simulink library "ASEToolBox"  (R2025b)
settings: Solver=ode45  StartTime=0.0  StopTime=10.0  RelTol=1e-3  EnableMultiTasking=on
values from neighbouring files (symbols this model uses):
  dt = get_param(gcbh, 'g_output_datatype')    [maskSysComCallbacks_Receive.m]    (also in maskSysComCallbacks_Send.m = get_param(gcbh, 'g_input_datatype'))
undefined symbols (not defined in the file or in its folder): dCx, dCy, dCz, DiscIntNeverNeededParam, Discrete, dmassX, dmassY, dmassZ, dMx, dMy, dMz, dp, dp0, dp1, dp2, dp3, dspblkCoreblockFVToolHelper, gcbh, lmd_high, lmd_low, magnitude, Newton, p0, p1, p2, p3, p4, phi0, phi000, phi1, phi2, phi3, phi4, r1, r2, r3, r4, Raphson, theta0, theta1, theta2, theta3, theta4, Time, u0, u1, u2, u3, v0, v0_max, v0_min, v1, v111, v2, v222, v3, v333, v4, W1, w1 ... (+4)
libraries: simulink x38, etargetslib x28, simulink_extras x5, slpidlib x2, ctrlSharedLib x2, aerolibatmos2 x1, aerolibconvert2 x1, aerolibtransform2 x1, sharedtransform x1, dspstat3 x1, dspsolvers x1
(part 3 of 6)

== system ASEToolBox/Aerocraft Model/ACE Aerodynamic for 3DOF/CL ==
  alpha : Inport
  Ma : Inport  Port=2
  deltz_pp : Inport  Port=3
  Add : Sum
  CL0 : Lookup2D  RowIndex=[-2,-1,0.5,1:10]  ColumnIndex=[0.3:0.1:0.8]  Table=|  SaturateOnIntegerOverflow=off  InputSameDT=off
      | [-0.8551	-0.8635	-0.8752	-0.8919	-0.914	-0.9479
      | -0.4232	-0.4273	-0.4332	-0.4415	-0.4525	-0.4695
      | 0.2105	0.2126	0.2155	0.2196	0.2251	0.2336
      | 0.4232	0.4273	0.4332	0.4415	0.4525	0.4695
      | 0.8551	0.8635	0.8752	0.8919	0.914	0.9479
      | 1.2956	1.3082	1.3258	1.351	1.3842	1.4353
      | 1.7443	1.7612	1.7848	1.8186	1.863	1.9315
      | 2.201	2.2223	2.2519	2.2944	2.3504	2.4364
      | 2.6653	2.691	2.7269	2.7783	2.846	2.95
      | 3.1369	3.1673	3.2096	3.2701	3.3498	3.4721
      | 3.6156	3.6507	3.6996	3.7695	3.8615	4.0026
      | 4.101	4.1411	4.1967	4.2764	4.381	4.5414
      | 4.593	4.6381	4.7008	4.7905	4.9082	5.0886
      | ]
  CLDeltZ : Lookup2D  RowIndex=|  ColumnIndex=|  Table=|  SaturateOnIntegerOverflow=off  InputSameDT=off
      RowIndex=|
      | [-2
      | -1
      | 0.5
      | 1
      | 2
      | 3
      | 4
      | 5
      | 6
      | 7
      | 8
      | 9
      | 10
      | ]
      Table=|
      | [0.0513	0.0522	0.0532	0.0541	0.0541	0.0541
      | 0.0513	0.0523	0.0532	0.0542	0.0542	0.0542
      | 0.0514	0.0523	0.0533	0.0542	0.0542	0.0542
      | 0.0513	0.0523	0.0532	0.0542	0.0542	0.0542
      | 0.0513	0.0522	0.0532	0.0541	0.0541	0.0541
      | 0.0512	0.0521	0.0531	0.054	0.054	0.054
      | 0.0511	0.052	0.053	0.0539	0.0539	0.0539
      | 0.0509	0.0518	0.0528	0.0537	0.0537	0.0537
      | 0.0507	0.0516	0.0526	0.0535	0.0535	0.0535
      | 0.0505	0.0514	0.0523	0.0533	0.0533	0.0533
      | 0.0502	0.0511	0.0521	0.053	0.053	0.053
      | 0.0499	0.0508	0.0517	0.0527	0.0527	0.0527
      | 0.0496	0.0505	0.0514	0.0523	0.0523	0.0523
      | ]
      ColumnIndex=|
      | [0.3	0.4	0.5	0.6	0.7	0.8
      | ]
  Divide1 : Product  Inputs=**
  CL : Outport
  wires:
  Add/1 -> CL/1
  Divide1/1 -> Add/2
  CL0/1 -> Add/1
  CLDeltZ/1 -> Divide1/2
  alpha/1 -> CL0/1, CLDeltZ/1
  Ma/1 -> CL0/2, CLDeltZ/2
  deltz_pp/1 -> Divide1/1

== system ASEToolBox/Aerocraft Model/ACE Aerodynamic for 3DOF/Subsystem1 ==
  beta : Inport
  alpha : Inport  Port=2
  Ma : Inport  Port=3
  CZBETA : Lookup2D  RowIndex=|  ColumnIndex=|  Table=|  SaturateOnIntegerOverflow=off  InputSameDT=off
      RowIndex=|
      | [-2
      | -1
      | 0.5
      | 1
      | 2
      | 3
      | 4
      | 5
      | 6
      | 7
      | 8
      | 9
      | 10
      | ]
      Table=|
      | [-0.3754	-0.3669	-0.3551	-0.3384	-0.3165	-0.2829
      | -0.3758	-0.3672	-0.3555	-0.3387	-0.3168	-0.2831
      | -0.3759	-0.3673	-0.3555	-0.3388	-0.3169	-0.2832
      | -0.3758	-0.3672	-0.3555	-0.3387	-0.3168	-0.2831
      | -0.3754	-0.3669	-0.3551	-0.3384	-0.3165	-0.2829
      | -0.3748	-0.3663	-0.3545	-0.3379	-0.316	-0.2824
      | -0.374	-0.3655	-0.3538	-0.3371	-0.3153	-0.2818
      | -0.3729	-0.3644	-0.3527	-0.3361	-0.3144	-0.281
      | -0.3716	-0.3631	-0.3515	-0.335	-0.3133	-0.2801
      | -0.37	-0.3616	-0.35	-0.3336	-0.312	-0.279
      | -0.3682	-0.3599	-0.3484	-0.332	-0.3106	-0.2777
      | -0.3662	-0.3579	-0.3465	-0.3302	-0.3089	-0.2762
      | -0.364	-0.3557	-0.3444	-0.3282	-0.3071	-0.2746
      | ]
      ColumnIndex=|
      | [0.3	0.4	0.5	0.6	0.7	0.8
      | ]
  Divide : Product  Inputs=**
  CZ : Outport
  wires:
  beta/1 -> Divide/1
  CZBETA/1 -> Divide/2
  Divide/1 -> CZ/1
  alpha/1 -> CZBETA/1
  Ma/1 -> CZBETA/2

== system ASEToolBox/Aerocraft Model/ACE Aerodynamic for 6DOF/CL Subsystem ==
  alpha : Inport
  Ma : Inport  Port=2
  DeltZ : Inport  Port=3
  Add : Sum
  CL0 : Lookup2D  RowIndex=[-2,-1,0.5,1:10]  ColumnIndex=[0.3:0.1:0.8]  Table=|  SaturateOnIntegerOverflow=off  InputSameDT=off
      | [-0.8551	-0.8635	-0.8752	-0.8919	-0.914	-0.9479
      | -0.4232	-0.4273	-0.4332	-0.4415	-0.4525	-0.4695
      | 0.2105	0.2126	0.2155	0.2196	0.2251	0.2336
      | 0.4232	0.4273	0.4332	0.4415	0.4525	0.4695
      | 0.8551	0.8635	0.8752	0.8919	0.914	0.9479
      | 1.2956	1.3082	1.3258	1.351	1.3842	1.4353
      | 1.7443	1.7612	1.7848	1.8186	1.863	1.9315
      | 2.201	2.2223	2.2519	2.2944	2.3504	2.4364
      | 2.6653	2.691	2.7269	2.7783	2.846	2.95
      | 3.1369	3.1673	3.2096	3.2701	3.3498	3.4721
      | 3.6156	3.6507	3.6996	3.7695	3.8615	4.0026
      | 4.101	4.1411	4.1967	4.2764	4.381	4.5414
      | 4.593	4.6381	4.7008	4.7905	4.9082	5.0886
      | ]
  CLDeltZ : Lookup2D  RowIndex=|  ColumnIndex=|  Table=|  SaturateOnIntegerOverflow=off  InputSameDT=off
      RowIndex=|
      | [-2
      | -1
      | 0.5
      | 1
      | 2
      | 3
      | 4
      | 5
      | 6
      | 7
      | 8
      | 9
      | 10
      | ]
      Table=|
      | [0.0513	0.0522	0.0532	0.0541	0.0541	0.0541
      | 0.0513	0.0523	0.0532	0.0542	0.0542	0.0542
      | 0.0514	0.0523	0.0533	0.0542	0.0542	0.0542
      | 0.0513	0.0523	0.0532	0.0542	0.0542	0.0542
      | 0.0513	0.0522	0.0532	0.0541	0.0541	0.0541
      | 0.0512	0.0521	0.0531	0.054	0.054	0.054
      | 0.0511	0.052	0.053	0.0539	0.0539	0.0539
      | 0.0509	0.0518	0.0528	0.0537	0.0537	0.0537
      | 0.0507	0.0516	0.0526	0.0535	0.0535	0.0535
      | 0.0505	0.0514	0.0523	0.0533	0.0533	0.0533
      | 0.0502	0.0511	0.0521	0.053	0.053	0.053
      | 0.0499	0.0508	0.0517	0.0527	0.0527	0.0527
      | 0.0496	0.0505	0.0514	0.0523	0.0523	0.0523
      | ]
      ColumnIndex=|
      | [0.3	0.4	0.5	0.6	0.7	0.8
      | ]
  Divide1 : Product  Inputs=**
  CL : Outport
  wires:
  DeltZ/1 -> Divide1/1
  Ma/1 -> CLDeltZ/2, CL0/2
  alpha/1 -> CLDeltZ/1, CL0/1
  CLDeltZ/1 -> Divide1/2
  CL0/1 -> Add/1
  Divide1/1 -> Add/2
  Add/1 -> CL/1

== system ASEToolBox/Aerocraft Model/ACE Aerodynamic for 6DOF/CZ Subsystem ==
  beta : Inport
  alpha : Inport  Port=2
  Ma : Inport  Port=3
  CZBETA : Lookup2D  RowIndex=|  ColumnIndex=|  Table=|  SaturateOnIntegerOverflow=off  InputSameDT=off
      RowIndex=|
      | [-2
      | -1
      | 0.5
      | 1
      | 2
      | 3
      | 4
      | 5
      | 6
      | 7
      | 8
      | 9
      | 10
      | ]
      Table=|
      | [-0.3754	-0.3669	-0.3551	-0.3384	-0.3165	-0.2829
      | -0.3758	-0.3672	-0.3555	-0.3387	-0.3168	-0.2831
      | -0.3759	-0.3673	-0.3555	-0.3388	-0.3169	-0.2832
      | -0.3758	-0.3672	-0.3555	-0.3387	-0.3168	-0.2831
      | -0.3754	-0.3669	-0.3551	-0.3384	-0.3165	-0.2829
      | -0.3748	-0.3663	-0.3545	-0.3379	-0.316	-0.2824
      | -0.374	-0.3655	-0.3538	-0.3371	-0.3153	-0.2818
      | -0.3729	-0.3644	-0.3527	-0.3361	-0.3144	-0.281
      | -0.3716	-0.3631	-0.3515	-0.335	-0.3133	-0.2801
      | -0.37	-0.3616	-0.35	-0.3336	-0.312	-0.279
      | -0.3682	-0.3599	-0.3484	-0.332	-0.3106	-0.2777
      | -0.3662	-0.3579	-0.3465	-0.3302	-0.3089	-0.2762
      | -0.364	-0.3557	-0.3444	-0.3282	-0.3071	-0.2746
      | ]
      ColumnIndex=|
      | [0.3	0.4	0.5	0.6	0.7	0.8
      | ]
  Divide : Product  Inputs=**
  CZ : Outport
  wires:
  Ma/1 -> CZBETA/2
  alpha/1 -> CZBETA/1
  Divide/1 -> CZ/1
  CZBETA/1 -> Divide/2
  beta/1 -> Divide/1

== system ASEToolBox/Aerocraft Model/ACE Aerodynamic for 6DOF/Mx Subsystem ==
  Beta : Inport
  Ma : Inport  Port=2
  alpha : Inport  Port=3
  DeltX : Inport  Port=4
  WX : Inport  Port=5
  WY : Inport  Port=6
  Add1 : Sum  Inputs=++++
  Divide{,2..4} (4 alike) : Product  Inputs=**
  MXBETA : Lookup2D  RowIndex=|  ColumnIndex=|  Table=|  SaturateOnIntegerOverflow=off  InputSameDT=off
      RowIndex=|
      | [-2
      | -1
      | 0.5
      | 1
      | 2
      | 3
      | 4
      | 5
      | 6
      | 7
      | 8
      | 9
      | 10
      | ]
      Table=|
      | [-0.0008	-0.0009	-0.0009	-0.0011	-0.0012	-0.0015
      | -0.0024	-0.0024	-0.0025	-0.0025	-0.0026	-0.0027
      | -0.0048	-0.0048	-0.0048	-0.0047	-0.0047	-0.0046
      | -0.0056	-0.0056	-0.0055	-0.0055	-0.0054	-0.0053
      | -0.0072	-0.0072	-0.0071	-0.0069	-0.0068	-0.0065
      | -0.0088	-0.0087	-0.0086	-0.0084	-0.0082	-0.0078
      | -0.0104	-0.0103	-0.0101	-0.0099	-0.0095	-0.009
      | -0.012	-0.0118	-0.0116	-0.0113	-0.0109	-0.0103
      | -0.0135	-0.0133	-0.0131	-0.0127	-0.0122	-0.0115
      | -0.015	-0.0148	-0.0145	-0.0141	-0.0135	-0.0127
      | -0.0165	-0.0163	-0.0159	-0.0155	-0.0148	-0.0139
      | -0.018	-0.0177	-0.0173	-0.0168	-0.0161	-0.015
      | -0.0194	-0.0191	-0.0187	-0.0181	-0.0174	-0.0162
      | ]
      ColumnIndex=|
      | [0.3	0.4	0.5	0.6	0.7	0.8
      | ]
  MXDeltX : Lookup2D  RowIndex=|  ColumnIndex=|  Table=|  SaturateOnIntegerOverflow=off  InputSameDT=off
      RowIndex=|
      | [-2
      | -1
      | 0.5
      | 1
      | 2
      | 3
      | 4
      | 5
      | 6
      | 7
      | 8
      | 9
      | 10
      | ]
      Table=|
      | [0.0035	0.0036	0.0037	0.0039	0.0042	0.0045
      | 0.0035	0.0036	0.0037	0.0039	0.0042	0.0045
      | 0.0035	0.0036	0.0037	0.0039	0.0042	0.0045
      | 0.0035	0.0036	0.0037	0.0039	0.0042	0.0045
      | 0.0035	0.0036	0.0037	0.0039	0.0042	0.0045
      | 0.0035	0.0036	0.0037	0.0039	0.0042	0.0045
      | 0.0034	0.0035	0.0037	0.0039	0.0042	0.0045
      | 0.0034	0.0035	0.0037	0.0039	0.0042	0.0045
      | 0.0034	0.0035	0.0037	0.0039	0.0042	0.0045
      | 0.0034	0.0035	0.0037	0.0039	0.0042	0.0045
      | 0.0034	0.0035	0.0037	0.0039	0.0041	0.0045
      | 0.0034	0.0035	0.0037	0.0039	0.0041	0.0045
      | 0.0034	0.0035	0.0037	0.0039	0.0041	0.0045
      | ]
      ColumnIndex=|
      | [0.3	0.4	0.5	0.6	0.7	0.8
      | ]
  MXWX : Lookup2D  RowIndex=|  ColumnIndex=|  Table=|  SaturateOnIntegerOverflow=off  InputSameDT=off
      RowIndex=|
      | [-2
      | -1
      | 0.5
      | 1
      | 2
      | 3
      | 4
      | 5
      | 6
      | 7
      | 8
      | 9
      | 10
      | ]
      Table=|
      | [-0.0034	-0.0033	-0.0033	-0.0031	-0.0031	-0.0032
      | -0.0037	-0.0036	-0.0035	-0.0033	-0.0033	-0.0034
      | -0.004	-0.004	-0.0039	-0.0037	-0.0036	-0.0036
      | -0.0041	-0.0041	-0.004	-0.0038	-0.0037	-0.0037
      | -0.0044	-0.0043	-0.0042	-0.0039	-0.0039	-0.0039
      | -0.0045	-0.0045	-0.0044	-0.0041	-0.0041	-0.004
      | -0.0047	-0.0046	-0.0045	-0.0043	-0.0042	-0.0041
      | -0.0048	-0.0047	-0.0046	-0.0044	-0.0043	-0.0042
      | -0.0049	-0.0048	-0.0047	-0.0045	-0.0044	-0.0043
      | -0.005	-0.0049	-0.0048	-0.0045	-0.0045	-0.0044
      | -0.0051	-0.005	-0.0049	-0.0046	-0.0045	-0.0044
      | -0.0051	-0.005	-0.0049	-0.0046	-0.0045	-0.0044
      | -0.0051	-0.005	-0.0049	-0.0046	-0.0045	-0.0044
      | ]
      ColumnIndex=|
      | [0.3	0.4	0.5	0.6	0.7	0.8
      | ]
  MXWY : Lookup2D  RowIndex=|  ColumnIndex=|  Table=|  SaturateOnIntegerOverflow=off  InputSameDT=off
      RowIndex=|
      | [-2
      | -1
      | 0.5
      | 1
      | 2
      | 3
      | 4
      | 5
      | 6
      | 7
      | 8
      | 9
      | 10
      | ]
      Table=|
      | [-0.0152	-0.0148	-0.0143	-0.0135	-0.0125	-0.011
      | -0.0146	-0.0143	-0.0138	-0.013	-0.0121	-0.0106
      | -0.0138	-0.0134	-0.013	-0.0123	-0.0114	-0.01
      | -0.0135	-0.0132	-0.0127	-0.012	-0.0112	-0.0099
      | -0.0129	-0.0126	-0.0122	-0.0115	-0.0107	-0.0095
      | -0.0123	-0.012	-0.0116	-0.011	-0.0103	-0.0091
      | -0.0117	-0.0115	-0.0111	-0.0105	-0.0098	-0.0087
      | -0.0112	-0.0109	-0.0105	-0.01	-0.0093	-0.0083
      | -0.0106	-0.0104	-0.01	-0.0095	-0.0089	-0.0079
      | -0.0101	-0.0098	-0.0095	-0.0091	-0.0085	-0.0076
      | -0.0095	-0.0093	-0.009	-0.0086	-0.008	-0.0072
      | -0.009	-0.0088	-0.0086	-0.0082	-0.0077	-0.0069
      | -0.0086	-0.0084	-0.0081	-0.0078	-0.0073	-0.0066
      | ]
      ColumnIndex=|
      | [0.3	0.4	0.5	0.6	0.7	0.8
      | ]
  Mx : Outport
  wires:
  Beta/1 -> Divide/2
  Ma/1 -> MXBETA/2, MXDeltX/2, MXWX/2, MXWY/2
  alpha/1 -> MXBETA/1, MXDeltX/1, MXWX/1, MXWY/1
  Add1/1 -> Mx/1
  Divide4/1 -> Add1/4
  Divide3/1 -> Add1/3
  Divide2/1 -> Add1/2
  Divide/1 -> Add1/1
  WY/1 -> Divide4/2
  MXWY/1 -> Divide4/1
  WX/1 -> Divide3/2
  MXWX/1 -> Divide3/1
  DeltX/1 -> Divide2/2
  MXDeltX/1 -> Divide2/1
  MXBETA/1 -> Divide/1

== system ASEToolBox/Aerocraft Model/ACE Aerodynamic for 6DOF/My Subsystem ==
  Beta : Inport
  WX : Inport  Port=2
  WY : Inport  Port=3
  Ma : Inport  Port=4
  alpha : Inport  Port=5
  Add2 : Sum  Inputs=+++
  Divide1 : Product  Inputs=**
  Divide2 : Product  Inputs=**
  Divide3 : Product  Inputs=**
  MYBETA : Lookup2D  RowIndex=|  ColumnIndex=|  Table=|  SaturateOnIntegerOverflow=off  InputSameDT=off
      RowIndex=|
      | [-2
      | -1
      | 0.5
      | 1
      | 2
      | 3
      | 4
      | 5
      | 6
      | 7
      | 8
      | 9
      | 10
      | ]
      Table=|
      | [-0.083	-0.0809	-0.078	-0.074	-0.0686	-0.0604
      | -0.0831	-0.081	-0.0781	-0.074	-0.0687	-0.0604
      | -0.083	-0.0809	-0.078	-0.0739	-0.0686	-0.0603
      | -0.0829	-0.0808	-0.078	-0.0739	-0.0685	-0.0603
      | -0.0827	-0.0806	-0.0778	-0.0737	-0.0683	-0.0601
      | -0.0824	-0.0803	-0.0775	-0.0734	-0.0681	-0.0599
      | -0.082	-0.08	-0.0771	-0.073	-0.0677	-0.0596
      | -0.0816	-0.0795	-0.0767	-0.0726	-0.0673	-0.0592
      | -0.081	-0.079	-0.0761	-0.0721	-0.0668	-0.0587
      | -0.0804	-0.0783	-0.0755	-0.0715	-0.0663	-0.0582
      | -0.0796	-0.0776	-0.0748	-0.0708	-0.0656	-0.0577
      | -0.0788	-0.0768	-0.074	-0.0701	-0.0649	-0.057
      | -0.0779	-0.0759	-0.0732	-0.0693	-0.0642	-0.0563
      | ]
      ColumnIndex=|
      | [0.3	0.4	0.5	0.6	0.7	0.8
      | ]
  MYWX : Lookup2D  RowIndex=|  ColumnIndex=|  Table=|  SaturateOnIntegerOverflow=off  InputSameDT=off
      RowIndex=|
      | [-2
      | -1
      | 0.5
      | 1
      | 2
      | 3
      | 4
      | 5
      | 6
      | 7
      | 8
      | 9
      | 10
      | ]
      Table=|
      | [-0.0014 	-0.0013 	-0.0013 	-0.0012 	-0.0011 	-0.0010 
      | -0.0007 	-0.0007 	-0.0006 	-0.0006 	-0.0006 	-0.0005 
      | 0.0003 	0.0003 	0.0003 	0.0003 	0.0003 	0.0002 
      | 0.0007 	0.0007 	0.0006 	0.0006 	0.0006 	0.0005 
      | 0.0014 	0.0013 	0.0013 	0.0012 	0.0011 	0.0010 
      | 0.0020 	0.0020 	0.0019 	0.0018 	0.0017 	0.0015 
      | 0.0027 	0.0026 	0.0025 	0.0024 	0.0022 	0.0019 
      | 0.0033 	0.0032 	0.0031 	0.0030 	0.0027 	0.0024 
      | 0.0039 	0.0038 	0.0037 	0.0035 	0.0032 	0.0028 
      | 0.0045 	0.0044 	0.0042 	0.0040 	0.0037 	0.0033 
      | 0.0050 	0.0049 	0.0047 	0.0045 	0.0041 	0.0036 
      | 0.0055 	0.0054 	0.0052 	0.0049 	0.0046 	0.0040 
      | 0.0060 	0.0058 	0.0056 	0.0053 	0.0049 	0.0043 
      | ]
      ColumnIndex=|
      | [0.3	0.4	0.5	0.6	0.7	0.8
      | ]
  MYWY : Lookup2D  RowIndex=|  ColumnIndex=|  Table=|  SaturateOnIntegerOverflow=off  InputSameDT=off
      RowIndex=|
      | [-2
      | -1
      | 0.5
      | 1
      | 2
      | 3
      | 4
      | 5
      | 6
      | 7
      | 8
      | 9
      | 10
      | ]
      Table=|
      | [-0.0401	-0.039	-0.0377	-0.0357	-0.0331	-0.0291
      | -0.0403	-0.0393	-0.0379	-0.0359	-0.0333	-0.0293
      | -0.0407	-0.0397	-0.0383	-0.0363	-0.0337	-0.0296
      | -0.0408	-0.0398	-0.0384	-0.0364	-0.0337	-0.0297
      | -0.041	-0.04	-0.0386	-0.0366	-0.0339	-0.0298
      | -0.0412	-0.0402	-0.0387	-0.0367	-0.0341	-0.03
      | -0.0414	-0.0403	-0.0389	-0.0369	-0.0342	-0.0301
      | -0.0415	-0.0404	-0.039	-0.037	-0.0343	-0.0302
      | -0.0416	-0.0405	-0.0391	-0.037	-0.0344	-0.0303
      | -0.0416	-0.0406	-0.0392	-0.0371	-0.0344	-0.0303
      | -0.0417	-0.0406	-0.0392	-0.0371	-0.0345	-0.0303
      | -0.0417	-0.0406	-0.0392	-0.0371	-0.0345	-0.0303
      | -0.0417	-0.0406	-0.0392	-0.0371	-0.0344	-0.0303
      | ]
      ColumnIndex=|
      | [0.3	0.4	0.5	0.6	0.7	0.8
      | ]
  My : Outport
  wires:
  WX/1 -> Divide3/2
  WY/1 -> Divide2/2
  Beta/1 -> Divide1/2
  Ma/1 -> MYBETA/2, MYWY/2, MYWX/2
  alpha/1 -> MYBETA/1, MYWY/1, MYWX/1
  Add2/1 -> My/1
  Divide3/1 -> Add2/3
  Divide2/1 -> Add2/2
  MYWX/1 -> Divide3/1
  MYWY/1 -> Divide2/1
  MYBETA/1 -> Divide1/1
  Divide1/1 -> Add2/1

== system ASEToolBox/Aerocraft Model/ACE Aerodynamic for 6DOF/Mz Subsystem ==
  Ma : Inport
  alpha : Inport  Port=2
  DeltZ : Inport  Port=3
  WZ : Inport  Port=4
  Add1 : Sum  Inputs=+++
  Divide2 : Product  Inputs=**
  Divide3 : Product  Inputs=**
  MZ0 : Lookup2D  RowIndex=[-2,-1,0.5,1,2,3,4,5,6,7,8,9,10]  ColumnIndex=[0.3,0.4,0.5,0.6,0.7,0.8]  Table=reshape([0.0795,0.0397,-0.0199,-0.0397,-0.0795,-0.1193,-0.1589,-0.1983,-0.2375,-0.2763,-0.3146,-0.3523,-0.3894,0.078,0.039,-0.0195,-0.039,-0.078,-0.117,-0.1558,-0.1945,-0.2329,-0.271,-0.3086,-0.3456,-0.382,0.0759,0.0379,-0.0189,-0.0379,-0.0759,-0.1138,-0.1516,-0.1892,-0.2266,-0.2637,-0.3003,-0.3364,-0.3718,0.0728,0.0364,-0.0182,-0.0364,-0.0728,-0.1092,-0.1455,-0.1816,-0.2175,-0.2531,-0.2883,-0.323,-0.3572,0.0687,0.0343,-0.0172,-0.0343,-0.0687,-0.1031,-0.1374,-0.1716,-0.2056,-0.2393,-0.2726,-0.3055,-0.3378,0.0624,0.0312,-0.0156,-0.0312,-0.0624,-0.0937,-0.1249,-0.1559,-0.1869,-0.2176,-0.248,-0.278,-0.3076],13,6)  SaturateOnIntegerOverflow=off  InputSameDT=off
  MZDeltZ : Lookup2D  RowIndex=|  ColumnIndex=|  Table=|  SaturateOnIntegerOverflow=off  InputSameDT=off
      RowIndex=|
      | [-2
      | -1
      | 0.5
      | 1
      | 2
      | 3
      | 4
      | 5
      | 6
      | 7
      | 8
      | 9
      | 10
      | ]
      Table=|
      | [0.0233	0.0237	0.0241	0.0246	0.0246	0.0246
      | 0.0233	0.0237	0.0242	0.0246	0.0246	0.0246
      | 0.0233	0.0237	0.0242	0.0246	0.0246	0.0246
      | 0.0233	0.0237	0.0242	0.0246	0.0246	0.0246
      | 0.0233	0.0237	0.0241	0.0246	0.0246	0.0246
      | 0.0232	0.0237	0.0241	0.0245	0.0245	0.0245
      | 0.0232	0.0236	0.024	0.0245	0.0245	0.0245
      | 0.0231	0.0235	0.024	0.0244	0.0244	0.0244
      | 0.023	0.0234	0.0239	0.0243	0.0243	0.0243
      | 0.0229	0.0233	0.0238	0.0242	0.0242	0.0242
      | 0.0228	0.0232	0.0236	0.0241	0.0241	0.0241
      | 0.0227	0.0231	0.0235	0.0239	0.0239	0.0239
      | 0.0225	0.0229	0.0233	0.0238	0.0238	0.0238
      | ]
      ColumnIndex=|
      | [0.3	0.4	0.5	0.6	0.7	0.8
      | ]
  MZWZ : Lookup2D  RowIndex=|  ColumnIndex=|  Table=|  SaturateOnIntegerOverflow=off  InputSameDT=off
      RowIndex=|
      | [-2
      | -1
      | 0.5
      | 1
      | 2
      | 3
      | 4
      | 5
      | 6
      | 7
      | 8
      | 9
      | 10
      | ]
      Table=|
      | [-0.0182	-0.0182	-0.0182	-0.0182	-0.0182	-0.0182
      | -0.0183	-0.0183	-0.0183	-0.0183	-0.0183	-0.0183
      | -0.0183	-0.0183	-0.0183	-0.0183	-0.0183	-0.0183
      | -0.0183	-0.0183	-0.0183	-0.0183	-0.0183	-0.0183
      | -0.0182	-0.0182	-0.0182	-0.0182	-0.0182	-0.0182
      | -0.0182	-0.0182	-0.0182	-0.0182	-0.0182	-0.0182
      | -0.0182	-0.0182	-0.0182	-0.0182	-0.0182	-0.0182
      | -0.0181	-0.0181	-0.0181	-0.0181	-0.0181	-0.0181
      | -0.018	-0.018	-0.018	-0.018	-0.018	-0.018
      | -0.018	-0.018	-0.018	-0.018	-0.018	-0.018
      | -0.0179	-0.0179	-0.0179	-0.0179	-0.0179	-0.0179
      | -0.0177	-0.0177	-0.0177	-0.0177	-0.0177	-0.0177
      | -0.0176	-0.0176	-0.0176	-0.0176	-0.0176	-0.0176
      | ]
      ColumnIndex=|
      | [0.3	0.4	0.5	0.6	0.7	0.8
      | ]
  Mz : Outport
  wires:
  DeltZ/1 -> Divide2/2
  MZDeltZ/1 -> Divide2/1
  WZ/1 -> Divide3/2
  Ma/1 -> MZ0/2, MZDeltZ/2, MZWZ/2
  alpha/1 -> MZ0/1, MZDeltZ/1, MZWZ/1
  MZWZ/1 -> Divide3/1
  Add1/1 -> Mz/1
  Divide3/1 -> Add1/3
  Divide2/1 -> Add1/2
  MZ0/1 -> Add1/1

== system ASEToolBox/Aerocraft Model/ACE Equation of 6DOF's Motion/ACE Centroid Motion ==
  note: deg
  P : Inport
  m : Inport  Port=2
  abv : Inport  Port=3
  F_aero : Inport  Port=4
  231 Motion Subsystem : Subsystem
  Calculate F_all : Subsystem
  Calculate xyz : Subsystem
  Demux2 : Demux  Outputs=3
  Gain1 : Gain  Gain=180/pi
  Gain2 : Gain  Gain=180/pi
  xyz : Outport
  theta : Outport  Port=2
  sigma : Outport  Port=3
  Vxyz : Outport  Port=4
  V : Outport  Port=5
  wires:
  231 Motion Subsystem/3(sigma) -> Calculate xyz/3(sigma), Gain2/1
  231 Motion Subsystem/1(V) -> Calculate xyz/1(V), V/1
  Calculate xyz/1(Vxyz) -> Vxyz/1
  Calculate xyz/2(xyz) -> xyz/1
  Gain2/1 -> sigma/1  "deg"
  Gain1/1 -> theta/1  "deg"
  231 Motion Subsystem/2(theta) -> Gain1/1, Calculate xyz/2(theta), Calculate F_all/7(Theta)
  P/1 -> Calculate F_all/1(P)
  F_aero/1 -> Calculate F_all/2(F_aero)
  m/1 -> Calculate F_all/3(m)
  Calculate F_all/1(F_All/m) -> 231 Motion Subsystem/1(F_All/m)
  abv/1 -> Demux2/1
  Demux2/1 -> Calculate F_all/4(alpha)
  Demux2/2 -> Calculate F_all/5(beta)
  Demux2/3 -> Calculate F_all/6(nu)

== system ASEToolBox/Aerocraft Model/ACE Equation of 6DOF's Motion/ACE Mass Properties ==
  Time : Inport
  Add : Sum  Inputs=|+++|
  Add1 : Sum  Inputs=+-
  Add2 : Sum  Inputs=+-
  Constant0 : Constant  Value=0
  Constant00 : Constant  Value=0
  Discrete-Time Integrator : DiscreteIntegrator  InitialConditionSource=external  SampleTime=-1  ICPrevOutput=DiscIntNeverNeededParam  ICPrevScaledInput=DiscIntNeverNeededParam
  Discrete-Time Integrator1 : DiscreteIntegrator  InitialConditionSource=external  SampleTime=-1  ICPrevOutput=DiscIntNeverNeededParam  ICPrevScaledInput=DiscIntNeverNeededParam
  Divide1 : Product  Inputs=/*
  Divide2 : Product  Inputs=/*
  Gain1 : Gain  Gain=-1
  Gain2 : Gain  Gain=-1
  Integrator1 : Integrator  Commented=on  InitialConditionSource=external
  Integrator3 : Integrator  Commented=on  InitialConditionSource=external
  Switch1 : Switch  SaturateOnIntegerOverflow=off  InputSameDT=off
  Switch2 : Switch  SaturateOnIntegerOverflow=off  InputSameDT=off
  Time1 : Constant  Value=6
  Time2 : Constant  Value=15
  m0 : Constant  Value=110
  m1 : Constant  Value=8
  m2 : Constant  Value=4
  m : Outport
  wires:
  Constant00/1 -> Switch2/1
  Discrete-Time Integrator1/1 -> Switch2/3
  Constant0/1 -> Switch1/1
  Discrete-Time Integrator/1 -> Switch1/3
  m1/1 -> Divide1/2, Discrete-Time Integrator/2
  m2/1 -> Divide2/2, Discrete-Time Integrator1/2
  Add/1 -> m/1
  Time1/1 -> Divide1/1, Add1/2
  Divide1/1 -> Gain1/1
  Gain1/1 -> Discrete-Time Integrator/1
  Time2/1 -> Divide2/1, Add2/2
  Divide2/1 -> Gain2/1
  Gain2/1 -> Discrete-Time Integrator1/1
  Time/1 -> Add1/1, Add2/1
  Switch1/1 -> Add/1
  Add1/1 -> Switch1/2
  Switch2/1 -> Add/3
  Add2/1 -> Switch2/2
  m0/1 -> Add/2

== system ASEToolBox/Aerocraft Model/ACE Equation of 6DOF's Motion/ACE Propulsion ==
  Time : Inport
  Add : Sum
  Add1 : Sum  Inputs=+-
  Add2 : Sum  Inputs=+-
  Constant0 : Constant  Value=0
  P1 : Constant  Value=3280
  P2 : Constant  Value=420
  Switch1 : Switch  SaturateOnIntegerOverflow=off  InputSameDT=off
  Switch2 : Switch  SaturateOnIntegerOverflow=off  InputSameDT=off
  Time1 : Constant  Value=6
  Time2 : Constant  Value=15
  P : Outport
  wires:
  Switch2/1 -> Switch1/1
  Add2/1 -> Switch2/2
  Constant0/1 -> Switch2/1
  Add1/1 -> Switch1/2
  Add/1 -> Switch1/3
  P1/1 -> Add/2
  P2/1 -> Add/1, Switch2/3
  Time2/1 -> Add2/2
  Time1/1 -> Add1/2
  Time/1 -> Add2/1, Add1/1
  Switch1/1 -> P/1

== system ASEToolBox/Aerocraft Model/ACE Equation of 6DOF's Motion/ACE Rotation Motion ==
  Mxyz : Inport
  Ixyz : Inport  Port=2
  "Attitude Dynamic " : Subsystem
  Eular0 : Constant  Value=[60 0 0]
  Wxyz : Gain  Gain=180/pi
  calculate Eular 231 : Subsystem
  Eular(deg) : Outport
  Wxyz1(deg/s) : Outport  Port=2
  wires:
  Eular0/1 -> calculate Eular 231/2(Eular0(deg))
  Ixyz/1 -> "Attitude Dynamic "/2(Ixyz)
  Wxyz/1 -> Wxyz1(deg/s)/1  "deg/s"
  "Attitude Dynamic "/1(Wxyz) -> calculate Eular 231/1(Wxyz), Wxyz/1  "rad/s"
  Mxyz/1 -> "Attitude Dynamic "/1(Mxyz)
  calculate Eular 231/1(Eular(deg)) -> Eular(deg)/1  "deg"

== system ASEToolBox/Aerocraft Model/ACE Equation of 6DOF's Motion/Aero Force & Moment ==
  H : Inport
  DeltXYZ : Inport  Port=2
  abv : Inport  Port=3
  V : Inport  Port=4
  Wxyz : Inport  Port=5
  ACE Aerodynamic for 6DOF : Subsystem  mask(ACE Aerodynamic for 6DOF){}
      mask help: There is ACE Aerodynamic for 6DOF Model, including the ACE aircraft's aerodynamic force efficient models and aerodynamic moment efficient models, and it is employed to simulate the 6DOF motion.
      mask Display:
      | image(imread('aeroaerodynamics.bmp','bmp'),'center')
      | port_label('input',1,'Mach(M)','texmode','on');
      | port_label('input',2,'abv(deg)','texmode','on');
      | port_label('input',3,'WXYZ','texmode','on');
      | port_label('input',4,'Deltaxyz(deg)','texmode','on');
      | port_label('output',1,'Cxyz','texmode','on');
      | port_label('output',2,'mxyz','texmode','on');
  Add4 : Sum
  COESA Atmosphere Model : aerolibatmos2/COESA Atmosphere Model  units=Metric (MKS)  spec=1976 COESA-extended U.S. Standard Atmosphere  model=Profile  profile_var=High temperature  profile_percent=1%  profile_alt=5 km (16404 ft)  envelope_var=High temperature  envelope_percent=1%  action=None
  Divide : Product  Inputs=/*  RndMeth=Zero
  L : Constant  Value=3
  Product1 : Product  Inputs=**  SaturateOnIntegerOverflow=on  OutDataTypeStr=Inherit: Same as first input
  Product2 : Product  Inputs=***  SaturateOnIntegerOverflow=on  OutDataTypeStr=Inherit: Same as first input
  Product8 : Product  Inputs=**/  InputSameDT=on  SaturateOnIntegerOverflow=on  OutDataTypeStr=Inherit: Same as first input
  Sm : Gain  Gain=0.0616
  Subsystem : Subsystem
  Terminator : Terminator
  Terminator1 : Terminator
  dCxyz : Gain  Gain=1+[dCx,dCy,dCz]
  dMxyz : Gain  Gain=1+[dMx,dMy,dMz]
  dmassXYZ : Constant  Value=[dmassX,dmassY,dmassZ]
  dp : Gain  Gain=1+dp
  q Subsystem : Subsystem
  F_aero : Outport
  Mxyz : Outport  Port=2
  static pressure : Outport  Port=3
  dynamic pressure : Outport  Port=4
  wires:
  dMxyz/1 -> Product2/2
  dCxyz/1 -> Product1/2
  dmassXYZ/1 -> Subsystem/2(dmassXYZ)
  dp/1 -> q Subsystem/2(Density)
  Add4/1 -> Mxyz/1
  Subsystem/1(dMxyz) -> Add4/1
  ACE Aerodynamic for 6DOF/2(Mxyz) -> dMxyz/1
  L/1 -> Product8/2, Product2/3, Subsystem/3(L)  "L"
  Wxyz/1 -> Product8/1
  Product2/1 -> Add4/2
  Product1/1 -> Subsystem/1(XYZ), F_aero/1
  V/1 -> Product8/3, q Subsystem/1(V), Divide/2  "v"
  H/1 -> COESA Atmosphere Model/1  "H"
  ACE Aerodynamic for 6DOF/1(Cxyz) -> dCxyz/1
  Sm/1 -> Product2/1, Product1/1
  abv/1 -> ACE Aerodynamic for 6DOF/2(abv)
  COESA Atmosphere Model/4 -> dp/1
  COESA Atmosphere Model/2 -> Divide/1  "a"
  COESA Atmosphere Model/1 -> Terminator/1
  q Subsystem/1(q) -> Sm/1, dynamic pressure/1
  Divide/1 -> ACE Aerodynamic for 6DOF/1(Ma)  "Mach"
  Product8/1 -> ACE Aerodynamic for 6DOF/3(WXYZ)  "WXYZ"
  DeltXYZ/1 -> ACE Aerodynamic for 6DOF/4(DeltXYZ)
  COESA Atmosphere Model/3 -> Terminator1/1, static pressure/1

== system ASEToolBox/Aerocraft Model/ACE Equation of 6DOF's Motion/Calculate H&S ==
  xyz : Inport
  Add : Sum
  Demux1 : Demux  Outputs=3
  H : Gain
  Math Function : Math  Operator=square  SignedPower=on
  Math Function1 : Math  Operator=square  SignedPower=on
  Range : Sqrt  AlgorithmType=Newton-Raphson
  H. : Outport
  S : Outport  Port=2
  wires:
  H/1 -> H./1
  Demux1/3 -> Math Function1/1
  Demux1/1 -> Math Function/1
  Demux1/2 -> H/1
  Range/1 -> S/1
  Add/1 -> Range/1
  Math Function1/1 -> Add/2
  Math Function/1 -> Add/1
  xyz/1 -> Demux1/1

== system ASEToolBox/Aerocraft Model/ACE Equation of 6DOF's Motion/Constraint Equation2 ==
  note: 231
      |
      | sin\beta = cos\theta * [ cos\gamma * sin(\psi - \sigma) + sin\phi * sin\gamma * cos(\psi - \sigma) ] - sin\theta * cos\phi * sin\gamma
      |
      | sin\alpha * cos\beta = cos\theta * [ sin\phi * cos\gamma * cos(\psi - \sigma) - sin\gamma * sin(\psi - \sigma) ] - sin\theta * cos\phi * cos\gamma
      |
      | sin\nu * cos\theta = cos\alpha * sin\beta * sin\phi - sin\alpha * sin\beta * cos\gamma * cos\phi + cos\beta * sin\gamma * cos\phi
      | .
  theta : Inport
  sigma : Inport  Port=2
  Eular : Inport  Port=3
  Alpha : Gain  Gain=180/pi
  Beta : Gain  Gain=180/pi
  Gain1 : Gain  Gain=pi/180
  Gain2 : Gain  Gain=pi/180
  Gain3 : Gain  Gain=pi/180
  Mux3 : Mux  Inputs=3
  Nu : Gain  Gain=180/pi
  alpha Subsystem : Subsystem
  beta Subsystem : Subsystem
  nu Subsystem : Subsystem
  abv : Outport
  wires:
  theta/1 -> Gain3/1
  sigma/1 -> Gain2/1
  beta Subsystem/1(beta) -> nu Subsystem/2(beta), alpha Subsystem/4(beta), Beta/1
  Eular/1 -> Gain1/1
  Gain3/1 -> beta Subsystem/1(theta), nu Subsystem/3(theta), alpha Subsystem/1(theta)
  Gain2/1 -> alpha Subsystem/2(sigma), beta Subsystem/2(sigma)
  Gain1/1 -> beta Subsystem/3(Eular), nu Subsystem/4(Eular), alpha Subsystem/3(Eular)
  alpha Subsystem/1(alpha) -> nu Subsystem/1(alpha), Alpha/1
  Nu/1 -> Mux3/3
  nu Subsystem/1(nu) -> Nu/1
  Mux3/1 -> abv/1
  Beta/1 -> Mux3/2
  Alpha/1 -> Mux3/1

== system ASEToolBox/SIMSystemModule/ASEMonitorIn/Enabled Subsystem ==
  in : Inport
  Enable : EnablePort
  out : Outport
  wires:
  in/1 -> out/1

== system ASEToolBox/SIMSystemModule/ASEMonitorIn/FrameCheck ==
  note: 判断前两个字节帧头、次两个字节帧长度、校验和
  In1 : Inport
  AND : Logic  Inputs=3  IconShape=distinctive  AllPortsSameDT=off  OutDataTypeStr=boolean
  Bitwise AND : simulink/Logic and Bit Operations/Bitwise Operator  logicop=AND  UseBitMask=on  BitMask=hex2dec('FF')  BitMaskRealWorld=Stored Integer
      settings: LibrarySourceBlock=|
      | simulink/Quick Insert/Logic and Bit
      | Operations/Bitwise AND
  Byte Unpack1 : etargetslib/Byte Unpack  dimensions={1}  datatypes={'uint16'}  byteAlign=1
      settings: LibrarySourceBlock=embeddedtargetslib/Host Communication/Byte Unpack
  Byte Unpack3 : etargetslib/Byte Unpack  dimensions={1}  datatypes={'uint16'}  byteAlign=1
      settings: LibrarySourceBlock=embeddedtargetslib/Host Communication/Byte Unpack
  Compare To Constant : simulink/Logic and Bit Operations/Compare To Constant  relop===  const=hex2dec('DAA5')  OutDataTypeStr=boolean
  Compare To Zero : simulink/Logic and Bit Operations/Compare To Zero  relop===  OutDataTypeStr=boolean
  Data Type Conversion : DataTypeConversion  OutDataTypeStr=uint32  SaturateOnIntegerOverflow=off  RndMeth=Floor
  Data Type Conversion1 : DataTypeConversion  OutDataTypeStr=uint8  SaturateOnIntegerOverflow=off  RndMeth=Floor
  Demux : Demux  Outputs=[2,2,-1]
      settings: DisplayOption=none
  Relational Operator : RelationalOperator  Operator===  OutDataTypeStr=boolean  RndMeth=Simplest  InputSameDT=off
  Sum ofElements : Sum  Inputs=+
  Terminator : Terminator
  Width : Width  DataType=uint16
  Out1 : Outport
  wires:
  AND/1 -> Out1/1
  Bitwise AND/1 -> Data Type Conversion1/1
  Demux/1 -> Byte Unpack3/1
  Compare To Constant/1 -> AND/1
  Compare To Zero/1 -> AND/3
  Width/1 -> Relational Operator/2
  Relational Operator/1 -> AND/2
  Demux/2 -> Byte Unpack1/1
  Byte Unpack1/1 -> Relational Operator/1
  In1/1 -> Demux/1, Data Type Conversion/1, Width/1
  Data Type Conversion/1 -> Sum ofElements/1
  Byte Unpack3/1 -> Compare To Constant/1
  Demux/3 -> Terminator/1
  Data Type Conversion1/1 -> Compare To Zero/1
  Sum ofElements/1 -> Bitwise AND/1

== system ASEToolBox/SIMSystemModule/ASEMonitorIn/Subsystem1 ==
  note: 除去帧头等12个字节之外的数据字节长度，如果为4的倍数则正常并解析为单精度，否则不进行解析（强行解析后报错）
  In1 : Inport
  Enable : EnablePort
  Byte Unpack3 : etargetslib/Byte Unpack  dimensions={1}  datatypes={'uint32'}  byteAlign=1
      settings: LibrarySourceBlock=embeddedtargetslib/Host Communication/Byte Unpack
  Compare To Zero : simulink/Logic and Bit Operations/Compare To Zero  relop===  OutDataTypeStr=boolean
  Constant : Constant  Value=4  OutDataTypeStr=uint16
  Data Type Conversion{,1..4} (5 alike) : DataTypeConversion  OutDataTypeStr=double  SaturateOnIntegerOverflow=off  RndMeth=Floor
  Demux : Demux  Outputs=[2,2,4,1,1,1,-1,1]
      settings: DisplayOption=none
  Mod : Math  Operator=mod
  Subsystem : Subsystem
  Terminator : Terminator
  Terminator1 : Terminator
  Terminator2 : Terminator
  Width : Width  DataType=uint16
  ACKFrameCounter : Outport
  ACKSourceID : Outport  Port=2
  ACKTargetID : Outport  Port=3
  ACKFrameType : Outport  Port=4
  ACKFramePara : Outport  Port=5
  wires:
  Constant/1 -> Mod/2
  Data Type Conversion3/1 -> ACKTargetID/1
  Demux/4 -> Data Type Conversion2/1
  In1/1 -> Demux/1
  Demux/8 -> Terminator/1
  Width/1 -> Mod/1
  Byte Unpack3/1 -> Data Type Conversion1/1
  Demux/3 -> Byte Unpack3/1
  Data Type Conversion4/1 -> ACKFrameType/1
  Data Type Conversion1/1 -> ACKFrameCounter/1
  Demux/6 -> Data Type Conversion4/1
  Demux/5 -> Data Type Conversion3/1
  Demux/2 -> Terminator1/1
  Demux/7 -> Subsystem/1(In1), Width/1
  Data Type Conversion2/1 -> ACKSourceID/1
  Demux/1 -> Terminator2/1
  Subsystem/1(Out1) -> Data Type Conversion/1
  Data Type Conversion/1 -> ACKFramePara/1
  Mod/1 -> Compare To Zero/1
  Compare To Zero/1 -> Subsystem/Enable

== system ASEToolBox/SIMSystemModule/ASEMonitorOut/BitCheckSum1 ==
  In1 : Inport
  Add : Sum
  Bitwise AND : simulink/Logic and Bit Operations/Bitwise Operator  logicop=AND  UseBitMask=on  BitMask=hex2dec('FF')  BitMaskRealWorld=Stored Integer
      settings: LibrarySourceBlock=|
      | simulink/Quick Insert/Logic and Bit
      | Operations/Bitwise AND
  Bitwise AND1 : simulink/Logic and Bit Operations/Bitwise Operator  logicop=AND  UseBitMask=on  BitMask=hex2dec('FF')  BitMaskRealWorld=Stored Integer
      settings: LibrarySourceBlock=|
      | simulink/Quick Insert/Logic and Bit
      | Operations/Bitwise AND
  Bitwise NOT : simulink/Logic and Bit Operations/Bitwise Operator  logicop=NOT  UseBitMask=off  BitMask=bin2dec('11011001')  BitMaskRealWorld=Stored Integer
      settings: LibrarySourceBlock=|
      | simulink/Quick Insert/Logic and Bit
      | Operations/Bitwise NOT
  Constant5 : Constant
  Data Type Conversion10 : DataTypeConversion  OutDataTypeStr=uint16  SaturateOnIntegerOverflow=off  RndMeth=Floor
  Data Type Conversion11 : DataTypeConversion  OutDataTypeStr=uint16  SaturateOnIntegerOverflow=off  RndMeth=Floor
  Data Type Conversion12 : DataTypeConversion  OutDataTypeStr=uint8  SaturateOnIntegerOverflow=off  RndMeth=Floor
  Data Type Conversion8 : DataTypeConversion  OutDataTypeStr=uint32  SaturateOnIntegerOverflow=off  RndMeth=Floor
  Sum of Elements : Sum  Inputs=+
  Out1 : Outport
  wires:
  Constant5/1 -> Data Type Conversion11/1
  Sum of Elements/1 -> Bitwise AND/1
  Bitwise AND/1 -> Data Type Conversion10/1
  Add/1 -> Bitwise AND1/1
  Bitwise NOT/1 -> Add/1
  Data Type Conversion11/1 -> Add/2
  Data Type Conversion8/1 -> Sum of Elements/1
  Data Type Conversion10/1 -> Bitwise NOT/1
  In1/1 -> Data Type Conversion8/1
  Data Type Conversion12/1 -> Out1/1
  Bitwise AND1/1 -> Data Type Conversion12/1

== system ASEToolBox/Subsystem/Formation-Control/Consistent formation control  ==
  u0_k : Inport
  X1_k_1 : Inport  Port=2
  X2_k_1 : Inport  Port=3
  X3_k_1 : Inport  Port=4
  X0_k_1 : Inport  Port=5
  Bus Creator : BusCreator  Inputs=4
  Bus Creator1 : BusCreator  Inputs=3
  Delay5 : Delay  DelayLength=1  InitialCondition=u0
  dp0 : Constant  Value=dp0
  dp1 : Constant  Value=dp1
  dp2 : Constant  Value=dp2
  dp3 : Constant  Value=dp3
  一致性控制——F1 : Subsystem
  一致性控制——F2 : Subsystem
  一致性控制——F3 : Subsystem
  u : Outport
  wires:
  X3_k_1/1 -> 一致性控制——F2/6(X3_k_1), 一致性控制——F3/6(X3_k_1)
  dp0/1 -> Bus Creator/1  "dp0"
  dp1/1 -> Bus Creator/2  "dp1"
  dp2/1 -> Bus Creator/3  "dp2"
  dp3/1 -> Bus Creator/4  "dp3"
  Bus Creator/1 -> [dp]
  u0_k/1 -> Delay5/1
  X0_k_1/1 -> 一致性控制——F1/2(X0_k_1), 一致性控制——F2/3(X0_k_1), 一致性控制——F3/3(X0_k_1)
  X1_k_1/1 -> 一致性控制——F1/3(X1_k_1), 一致性控制——F2/4(X1_k_1), 一致性控制——F3/4(X1_k_1)
  X2_k_1/1 -> 一致性控制——F2/5(X2_k_1), 一致性控制——F3/5(X2_k_1), 一致性控制——F1/4(X2_k_1)
  一致性控制——F1/1(u1_k) -> [u1_k]
  [dp] -> 一致性控制——F3/1(dp), 一致性控制——F2/1(dp), 一致性控制——F1/5(dp)
  一致性控制——F2/1(u2_k) -> [u2_k]
  一致性控制——F3/1(u3_k) -> [u3_k]
  [u1_k] -> Bus Creator1/1  "u1_k"
  [u2_k] -> Bus Creator1/2  "u2_k"
  [u3_k] -> Bus Creator1/3  "u3_k"
  Bus Creator1/1 -> u/1
  Delay5/1 -> 一致性控制——F1/1(u0_k), 一致性控制——F3/2(u0_k), 一致性控制——F2/2(u0_k)

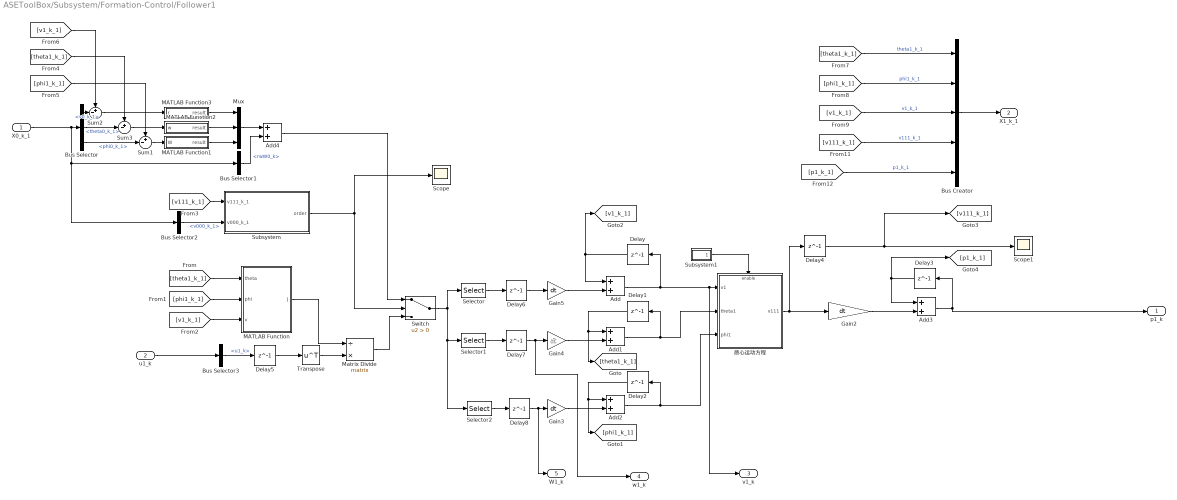
== system ASEToolBox/Subsystem/Formation-Control/Follower1 ==
  note: dt
  X0_k_1 : Inport
  u1_k : Inport  Port=2
  Add{,1..4} (5 alike) : Sum
  Bus Creator : BusCreator  Inputs=5
  Bus Selector : BusSelector  OutputSignals=v0_k_1,theta0_k_1,phi0_k_1
  Bus Selector1 : BusSelector  OutputSignals=rwW0_k
  Bus Selector2 : BusSelector  OutputSignals=v000_k_1
  Bus Selector3 : BusSelector  OutputSignals=u1_k
  Delay : Delay  DelayLength=1  InitialCondition=v1
  Delay1 : Delay  DelayLength=1  InitialCondition=theta1
  Delay2 : Delay  DelayLength=1  InitialCondition=phi1
  Delay3 : Delay  DelayLength=1  InitialCondition=p1
  Delay4 : Delay  DelayLength=1  InitialCondition=v111
  Delay5 : Delay  DelayLength=1  InitialCondition=u1
  Delay6 : Delay  DelayLength=1  InitialCondition=r1
  Delay7 : Delay  DelayLength=1  InitialCondition=w1
  Delay8 : Delay  DelayLength=1  InitialCondition=W1
  Gain{2..5} (4 alike) : Gain  Gain=dt
  MATLAB Function : MATLAB Function  TreatAsAtomicUnit=on
  MATLAB Function1 : MATLAB Function  TreatAsAtomicUnit=on
  MATLAB Function2 : MATLAB Function  TreatAsAtomicUnit=on
  MATLAB Function3 : MATLAB Function  TreatAsAtomicUnit=on
  Matrix Divide : Product  Inputs=/*  Multiplication=Matrix(*)
  Mux : Mux  Inputs=3
  Scope : Scope
      settings: ActiveDisplayYMinimum=-0.125  ActiveDisplayYMaximum=1.125
  Scope1 : Scope
      settings: ActiveDisplayYMinimum=-0.00358  ActiveDisplayYMaximum=0.0004
  Selector : Selector  InputPortWidth=3  IndexOptions=Index vector (dialog)  Indices=[1]  OutputSizes=1
  Selector1 : Selector  InputPortWidth=3  IndexOptions=Index vector (dialog)  Indices=[2]  OutputSizes=1
  Selector2 : Selector  InputPortWidth=3  IndexOptions=Index vector (dialog)  Indices=[3]  OutputSizes=1
  Subsystem : Subsystem
  Subsystem1 : Subsystem
  Sum1 : Sum  Inputs=+-|
  Sum2 : Sum  Inputs=+-|
  Sum3 : Sum  Inputs=+-|
  Switch : Switch  Criteria=u2 > Threshold  SaturateOnIntegerOverflow=off  InputSameDT=off
  Transpose : Math  Operator=transpose
  质心运动方程 : Subsystem
  p1_k : Outport
  X1_k_1 : Outport  Port=2
  v1_k : Outport  Port=3
  w1_k : Outport  Port=4
  W1_k : Outport  Port=5
  wires:
  [v1_k_1] -> MATLAB Function/3(v)
  [phi1_k_1] -> MATLAB Function/2(phi)
  [theta1_k_1] -> MATLAB Function/1(theta)
  Gain4/1 -> Add1/2
  Gain3/1 -> Add2/2
  Switch/1 -> Selector2/1, Selector1/1, Selector/1
  Delay3/1 -> Add3/1, [p1_k_1]
  Gain2/1 -> Add3/2
  Delay2/1 -> [phi1_k_1], Add2/1
  Add2/1 -> 质心运动方程/3(phi1), Delay2/1
  Add1/1 -> 质心运动方程/2(theta1), Delay1/1
  Delay/1 -> Add/1, [v1_k_1]
  Add/1 -> v1_k/1, 质心运动方程/1(v1), Delay/1
  Gain5/1 -> Add/2
  MATLAB Function/1(J) -> Matrix Divide/1
  u1_k/1 -> Bus Selector3/1
  Selector/1 -> Delay6/1
  Selector1/1 -> Delay7/1
  Selector2/1 -> Delay8/1
  Subsystem/1(order) -> Switch/2, Scope/1
  Matrix Divide/1 -> Switch/3
  质心运动方程/1(v111) -> Delay4/1, Gain2/1
  [v111_k_1] -> Subsystem/1(v111_k_1)
  Bus Selector2/1 -> Subsystem/2(v000_k_1)  "<v000_k_1>"
  X0_k_1/1 -> Bus Selector2/1, Bus Selector1/1, Bus Selector/1
  Bus Selector1/1 -> Add4/2  "<rwW0_k>"
  MATLAB Function2/1(result) -> Mux/2
  MATLAB Function1/1(result) -> Mux/3
  MATLAB Function3/1(result) -> Mux/1
  Mux/1 -> Add4/1
  Bus Selector/2 -> Sum3/2  "<theta0_k_1>"
  Sum3/1 -> MATLAB Function2/1(w)
  Bus Selector/3 -> Sum1/2  "<phi0_k_1>"
  Bus Selector/1 -> Sum2/2  "<v0_k_1>"
  Sum2/1 -> MATLAB Function3/1(r)
  Sum1/1 -> MATLAB Function1/1(W)
  [theta1_k_1] -> Sum3/1
  [phi1_k_1] -> Sum1/1
  [v1_k_1] -> Sum2/1
  [v111_k_1] -> Bus Creator/4  "v111_k_1"
  [p1_k_1] -> Bus Creator/5  "p1_k_1"
  [v1_k_1] -> Bus Creator/3  "v1_k_1"
  Bus Creator/1 -> X1_k_1/1
  [phi1_k_1] -> Bus Creator/2  "phi1_k_1"
  [theta1_k_1] -> Bus Creator/1  "theta1_k_1"
  Delay5/1 -> Transpose/1
  Add4/1 -> Switch/1
  Delay6/1 -> Gain5/1
  Delay7/1 -> w1_k/1, Gain4/1
  Delay8/1 -> W1_k/1, Gain3/1
  Delay4/1 -> [v111_k_1], Scope1/1
  Bus Selector3/1 -> Delay5/1  "<u1_k>"
  Transpose/1 -> Matrix Divide/2
  Delay1/1 -> [theta1_k_1], Add1/1
  Add3/1 -> p1_k/1, Delay3/1
  Subsystem1/1(Out1) -> 质心运动方程/Enable

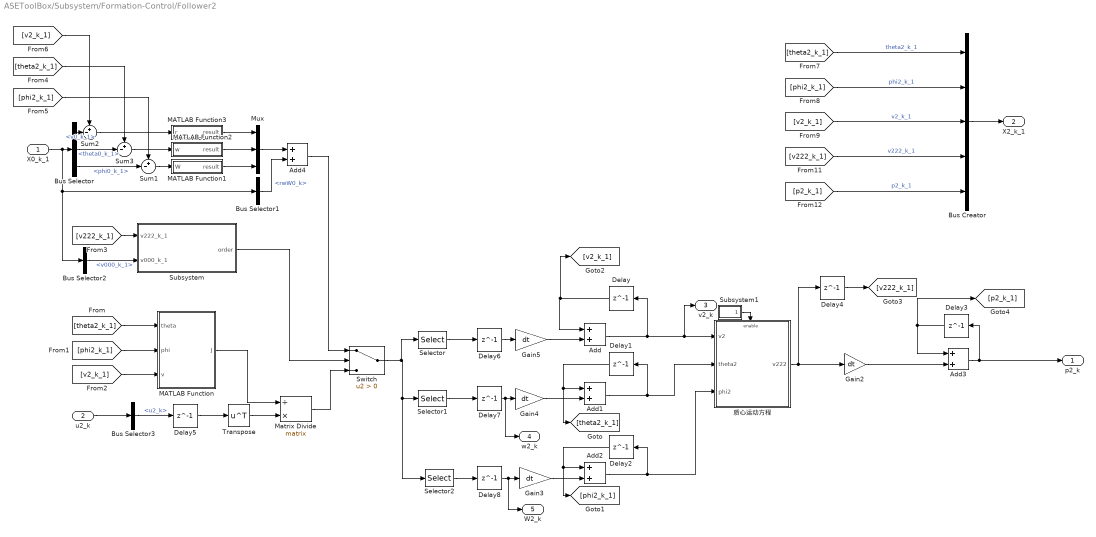
== system ASEToolBox/Subsystem/Formation-Control/Follower2 ==
  X0_k_1 : Inport
  u2_k : Inport  Port=2
  Add{,1..4} (5 alike) : Sum
  Bus Creator : BusCreator  Inputs=5
  Bus Selector : BusSelector  OutputSignals=v0_k_1,theta0_k_1,phi0_k_1
  Bus Selector1 : BusSelector  OutputSignals=rwW0_k
  Bus Selector2 : BusSelector  OutputSignals=v000_k_1
  Bus Selector3 : BusSelector  OutputSignals=u2_k
  Delay : Delay  DelayLength=1  InitialCondition=v2
  Delay1 : Delay  DelayLength=1  InitialCondition=theta2
  Delay2 : Delay  DelayLength=1  InitialCondition=phi2
  Delay3 : Delay  DelayLength=1  InitialCondition=p2
  Delay4 : Delay  DelayLength=1  InitialCondition=v222
  Delay5 : Delay  DelayLength=1  InitialCondition=u2
  Delay6 : Delay  DelayLength=1  InitialCondition=w2
  Delay7 : Delay  DelayLength=1  InitialCondition=W2
  Delay8 : Delay  DelayLength=1  InitialCondition=r2
  Gain{2..5} (4 alike) : Gain  Gain=dt
  MATLAB Function : MATLAB Function  TreatAsAtomicUnit=on
  MATLAB Function1 : MATLAB Function  TreatAsAtomicUnit=on
  MATLAB Function2 : MATLAB Function  TreatAsAtomicUnit=on
  MATLAB Function3 : MATLAB Function  TreatAsAtomicUnit=on
  Matrix Divide : Product  Inputs=/*  Multiplication=Matrix(*)
  Mux : Mux  Inputs=3
  Selector : Selector  InputPortWidth=3  IndexOptions=Index vector (dialog)  Indices=[1]  OutputSizes=1
  Selector1 : Selector  InputPortWidth=3  IndexOptions=Index vector (dialog)  Indices=[2]  OutputSizes=1
  Selector2 : Selector  InputPortWidth=3  IndexOptions=Index vector (dialog)  Indices=[3]  OutputSizes=1
  Subsystem : Subsystem
  Subsystem1 : Subsystem
  Sum1 : Sum  Inputs=+-|
  Sum2 : Sum  Inputs=+-|
  Sum3 : Sum  Inputs=+-|
  Switch : Switch  Criteria=u2 > Threshold  SaturateOnIntegerOverflow=off  InputSameDT=off
  Transpose : Math  Operator=transpose
  质心运动方程 : Subsystem
  p2_k : Outport
  X2_k_1 : Outport  Port=2
  v2_k : Outport  Port=3
  w2_k : Outport  Port=4
  W2_k : Outport  Port=5
  wires:
  [theta2_k_1] -> Bus Creator/1  "theta2_k_1"
  [phi2_k_1] -> Bus Creator/2  "phi2_k_1"
  Bus Creator/1 -> X2_k_1/1
  [v2_k_1] -> Bus Creator/3  "v2_k_1"
  [p2_k_1] -> Bus Creator/5  "p2_k_1"
  [v222_k_1] -> Bus Creator/4  "v222_k_1"
  [v2_k_1] -> Sum2/1
  [phi2_k_1] -> Sum1/1
  [theta2_k_1] -> Sum3/1
  Sum1/1 -> MATLAB Function1/1(W)
  Sum2/1 -> MATLAB Function3/1(r)
  Bus Selector/1 -> Sum2/2  "<v0_k_1>"
  Bus Selector/3 -> Sum1/2  "<phi0_k_1>"
  Sum3/1 -> MATLAB Function2/1(w)
  Bus Selector/2 -> Sum3/2  "<theta0_k_1>"
  Mux/1 -> Add4/1
  MATLAB Function3/1(result) -> Mux/1
  MATLAB Function1/1(result) -> Mux/3
  MATLAB Function2/1(result) -> Mux/2
  Bus Selector1/1 -> Add4/2  "<rwW0_k>"
  X0_k_1/1 -> Bus Selector/1, Bus Selector1/1, Bus Selector2/1
  Bus Selector2/1 -> Subsystem/2(v000_k_1)  "<v000_k_1>"
  [v222_k_1] -> Subsystem/1(v222_k_1)
  Matrix Divide/1 -> Switch/3
  Subsystem/1(order) -> Switch/2
  Add4/1 -> Switch/1
  Selector2/1 -> Delay8/1
  Selector1/1 -> Delay7/1
  Selector/1 -> Delay6/1
  u2_k/1 -> Bus Selector3/1
  MATLAB Function/1(J) -> Matrix Divide/1
  Gain5/1 -> Add/2
  Add/1 -> Delay/1, v2_k/1, 质心运动方程/1(v2)
  Delay/1 -> [v2_k_1], Add/1
  Delay1/1 -> [theta2_k_1], Add1/1
  Add1/1 -> 质心运动方程/2(theta2), Delay1/1
  Add2/1 -> 质心运动方程/3(phi2), Delay2/1
  Delay2/1 -> [phi2_k_1], Add2/1
  质心运动方程/1(v222) -> Gain2/1, Delay4/1
  Gain2/1 -> Add3/2
  Switch/1 -> Selector/1, Selector1/1, Selector2/1
  Gain3/1 -> Add2/2
  Gain4/1 -> Add1/2
  [theta2_k_1] -> MATLAB Function/1(theta)
  [phi2_k_1] -> MATLAB Function/2(phi)
  [v2_k_1] -> MATLAB Function/3(v)
  Delay5/1 -> Transpose/1
  Delay6/1 -> Gain5/1
  Delay7/1 -> w2_k/1, Gain4/1
  Delay8/1 -> W2_k/1, Gain3/1
  Bus Selector3/1 -> Delay5/1  "<u2_k>"
  Transpose/1 -> Matrix Divide/2
  Add3/1 -> Delay3/1, p2_k/1
  Delay3/1 -> [p2_k_1], Add3/1
  Delay4/1 -> [v222_k_1]
  Subsystem1/1(Out1) -> 质心运动方程/Enable

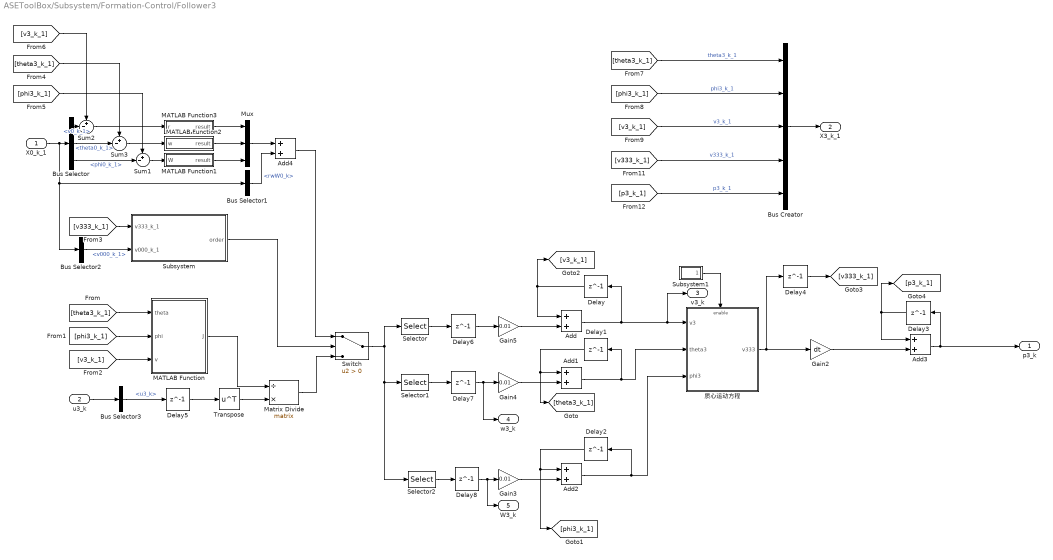
== system ASEToolBox/Subsystem/Formation-Control/Follower3 ==
  X0_k_1 : Inport
  u3_k : Inport  Port=2
  Add{,1..4} (5 alike) : Sum
  Bus Creator : BusCreator  Inputs=5
  Bus Selector : BusSelector  OutputSignals=v0_k_1,theta0_k_1,phi0_k_1
  Bus Selector1 : BusSelector  OutputSignals=rwW0_k
  Bus Selector2 : BusSelector  OutputSignals=v000_k_1
  Bus Selector3 : BusSelector  OutputSignals=u3_k
  Delay : Delay  DelayLength=1  InitialCondition=v3
  Delay1 : Delay  DelayLength=1  InitialCondition=theta3
  Delay2 : Delay  DelayLength=1  InitialCondition=phi3
  Delay3 : Delay  DelayLength=1  InitialCondition=p3
  Delay4 : Delay  DelayLength=1  InitialCondition=v333
  Delay5 : Delay  DelayLength=1  InitialCondition=u3
  Delay6 : Delay  DelayLength=1  InitialCondition=r3
  Delay7 : Delay  DelayLength=1  InitialCondition=w3
  Delay8 : Delay  DelayLength=1  InitialCondition=W3
  Gain2 : Gain  Gain=dt
  Gain3 : Gain  Gain=0.01
  Gain4 : Gain  Gain=0.01
  Gain5 : Gain  Gain=0.01
  MATLAB Function : MATLAB Function  TreatAsAtomicUnit=on
  MATLAB Function1 : MATLAB Function  TreatAsAtomicUnit=on
  MATLAB Function2 : MATLAB Function  TreatAsAtomicUnit=on
  MATLAB Function3 : MATLAB Function  TreatAsAtomicUnit=on
  Matrix Divide : Product  Inputs=/*  Multiplication=Matrix(*)
  Mux : Mux  Inputs=3
  Selector : Selector  InputPortWidth=3  IndexOptions=Index vector (dialog)  Indices=[1]  OutputSizes=1
  Selector1 : Selector  InputPortWidth=3  IndexOptions=Index vector (dialog)  Indices=[2]  OutputSizes=1
  Selector2 : Selector  InputPortWidth=3  IndexOptions=Index vector (dialog)  Indices=[3]  OutputSizes=1
  Subsystem : Subsystem
  Subsystem1 : Subsystem
  Sum1 : Sum  Inputs=+-|
  Sum2 : Sum  Inputs=+-|
  Sum3 : Sum  Inputs=+-|
  Switch : Switch  Criteria=u2 > Threshold  SaturateOnIntegerOverflow=off  InputSameDT=off
  Transpose : Math  Operator=transpose
  质心运动方程 : Subsystem
  p3_k : Outport
  X3_k_1 : Outport  Port=2
  v3_k : Outport  Port=3
  w3_k : Outport  Port=4
  W3_k : Outport  Port=5
  wires:
  [v3_k_1] -> MATLAB Function/3(v)
  [phi3_k_1] -> MATLAB Function/2(phi)
  [theta3_k_1] -> MATLAB Function/1(theta)
  Gain4/1 -> Add1/2
  Gain3/1 -> Add2/2
  Switch/1 -> Selector1/1, Selector2/1, Selector/1
  Delay3/1 -> [p3_k_1], Add3/1
  Gain2/1 -> Add3/2
  质心运动方程/1(v333) -> Delay4/1, Gain2/1
  Delay2/1 -> [phi3_k_1], Add2/1
  Add2/1 -> Delay2/1, 质心运动方程/3(phi3)
  Add1/1 -> 质心运动方程/2(theta3), Delay1/1
  Delay1/1 -> Add1/1, [theta3_k_1]
  Delay/1 -> Add/1, [v3_k_1]
  Add/1 -> Delay/1, v3_k/1, 质心运动方程/1(v3)
  Gain5/1 -> Add/2
  MATLAB Function/1(J) -> Matrix Divide/1
  u3_k/1 -> Bus Selector3/1
  Selector/1 -> Delay6/1
  Selector1/1 -> Delay7/1
  Selector2/1 -> Delay8/1
  Add4/1 -> Switch/1
  Subsystem/1(order) -> Switch/2
  Matrix Divide/1 -> Switch/3
  [v333_k_1] -> Subsystem/1(v333_k_1)
  Bus Selector2/1 -> Subsystem/2(v000_k_1)  "<v000_k_1>"
  X0_k_1/1 -> Bus Selector2/1, Bus Selector1/1, Bus Selector/1
  Bus Selector1/1 -> Add4/2  "<rwW0_k>"
  MATLAB Function2/1(result) -> Mux/2
  MATLAB Function1/1(result) -> Mux/3
  MATLAB Function3/1(result) -> Mux/1
  Mux/1 -> Add4/1
  Bus Selector/2 -> Sum3/2  "<theta0_k_1>"
  Sum3/1 -> MATLAB Function2/1(w)
  Bus Selector/3 -> Sum1/2  "<phi0_k_1>"
  Bus Selector/1 -> Sum2/2  "<v0_k_1>"
  Sum2/1 -> MATLAB Function3/1(r)
  Sum1/1 -> MATLAB Function1/1(W)
  [theta3_k_1] -> Sum3/1
  [phi3_k_1] -> Sum1/1
  [v3_k_1] -> Sum2/1
  [v333_k_1] -> Bus Creator/4  "v333_k_1"
  [p3_k_1] -> Bus Creator/5  "p3_k_1"
  [v3_k_1] -> Bus Creator/3  "v3_k_1"
  Bus Creator/1 -> X3_k_1/1
  [phi3_k_1] -> Bus Creator/2  "phi3_k_1"
  [theta3_k_1] -> Bus Creator/1  "theta3_k_1"
  Delay6/1 -> Gain5/1
  Delay7/1 -> w3_k/1, Gain4/1
  Delay8/1 -> W3_k/1, Gain3/1
  Delay5/1 -> Transpose/1
  Bus Selector3/1 -> Delay5/1  "<u3_k>"
  Transpose/1 -> Matrix Divide/2
  Add3/1 -> p3_k/1, Delay3/1
  Delay4/1 -> [v333_k_1]
  Subsystem1/1(Out1) -> 质心运动方程/Enable

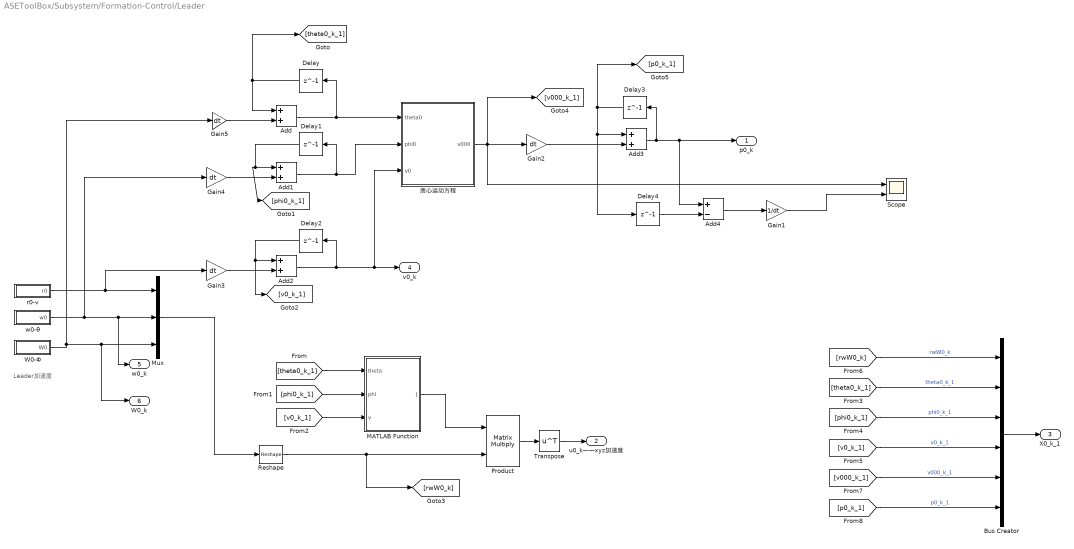
== system ASEToolBox/Subsystem/Formation-Control/Leader ==
  note: Leader加速度
  Add{,1..3} (4 alike) : Sum
  Add4 : Sum  Inputs=+-
  Bus Creator : BusCreator  Inputs=6
  Delay : Delay  DelayLength=1  InitialCondition=theta0
  Delay1 : Delay  DelayLength=1  InitialCondition=phi0
  Delay2 : Delay  DelayLength=1  InitialCondition=v0
  Delay3 : Delay  DelayLength=1  InitialCondition=p0
  Delay4 : Delay  DelayLength=1  InitialCondition=p0
  Gain1 : Gain  Gain=1/dt
  Gain{2..5} (4 alike) : Gain  Gain=dt
  MATLAB Function : MATLAB Function  TreatAsAtomicUnit=on
  Mux : Mux  Inputs=3
  Product : Product  Multiplication=Matrix(*)
  Reshape : Reshape  OutputDimensionality=Customize  OutputDimensions=[3,1]
  Scope : Scope  NumInputPorts=2
      settings: ActiveDisplayYMinimum=-3.73518  ActiveDisplayYMaximum=3.7362
  Transpose : Math  Operator=transpose
  W0-Φ : Subsystem
  r0-v : Subsystem
  w0-θ : Subsystem
  质心运动方程 : Subsystem
  p0_k : Outport
  u0_k——xyz加速度 : Outport  Port=2
  X0_k_1 : Outport  Port=3
  v0_k : Outport  Port=4
  w0_k : Outport  Port=5
  W0_k : Outport  Port=6
  wires:
  MATLAB Function/1(J) -> Product/1
  Mux/1 -> Reshape/1
  Gain5/1 -> Add/2
  Add/1 -> Delay/1, 质心运动方程/1(theta0)
  Delay/1 -> [theta0_k_1], Add/1
  w0-θ/1(w0) -> Gain4/1, w0_k/1, Mux/2
  Delay1/1 -> Add1/1, [phi0_k_1]
  Add1/1 -> Delay1/1, 质心运动方程/2(phi0)
  r0-v/1(r0) -> Gain3/1, Mux/1
  Add2/1 -> Delay2/1, 质心运动方程/3(v0), v0_k/1
  Delay2/1 -> Add2/1, [v0_k_1]
  Gain2/1 -> Add3/2
  Add3/1 -> Delay3/1, Add4/1, p0_k/1
  Delay3/1 -> [p0_k_1], Delay4/1, Add3/1
  Gain3/1 -> Add2/2
  Gain4/1 -> Add1/2
  W0-Φ/1(W0) -> Gain5/1, W0_k/1, Mux/3
  Reshape/1 -> [rwW0_k], Product/2
  [theta0_k_1] -> MATLAB Function/1(theta)
  [phi0_k_1] -> MATLAB Function/2(phi)
  [v0_k_1] -> MATLAB Function/3(v)
  [theta0_k_1] -> Bus Creator/2  "theta0_k_1"
  [phi0_k_1] -> Bus Creator/3  "phi0_k_1"
  [v0_k_1] -> Bus Creator/4  "v0_k_1"
  [rwW0_k] -> Bus Creator/1  "rwW0_k"
  Bus Creator/1 -> X0_k_1/1
  [v000_k_1] -> Bus Creator/5  "v000_k_1"
  [p0_k_1] -> Bus Creator/6  "p0_k_1"
  质心运动方程/1(v000) -> [v000_k_1], Scope/1, Gain2/1
  Product/1 -> Transpose/1
  Transpose/1 -> u0_k——xyz加速度/1
  Add4/1 -> Gain1/1
  Gain1/1 -> Scope/2
  Delay4/1 -> Add4/2
